simulink model "BlocoHidraulicoLAC_closeLoop"  (R2026a)
settings: Solver=ode15s  StopTime=5  FixedStep=0.001  MaxStep=1e-4
values from neighbouring files (symbols this model uses):
  Gamma = sys_d.B    [sintese_lqi_luenberger_lac.m]    (also in sintese_lqi_luenberger_lac_bateria_de_ensaio.m)
  K_i = -K_aug(3)    [sintese_lqi_luenberger_lac.m]    (also in sintese_lqi_luenberger_lac_bateria_de_ensaio.m)
  K_lqr = [K_pos, K_vel]    [sintese_lqi_luenberger_lac.m]    (also in sintese_lqi_luenberger_lac_bateria_de_ensaio.m)
  L_obs = place(Phi', Cx', polos_obs)'    [sintese_lqi_luenberger_lac.m]    (also in sintese_lqi_luenberger_lac_bateria_de_ensaio.m)
  Phi = sys_d.A    [sintese_lqi_luenberger_lac.m]    (also in sintese_lqi_luenberger_lac_bateria_de_ensaio.m)
undefined symbols (not defined in the file or in its folder): sigbuilder_block
(part 1 of 4)
settings Model: Creator=uidq5744  LastModifiedBy=uidq5744

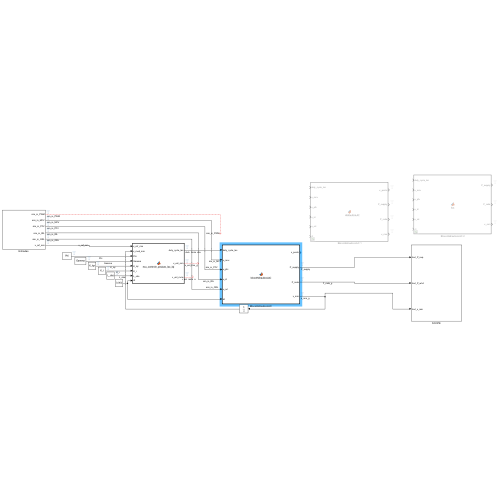
[thumbnail: Simulink's stored preview of the top-level diagram]
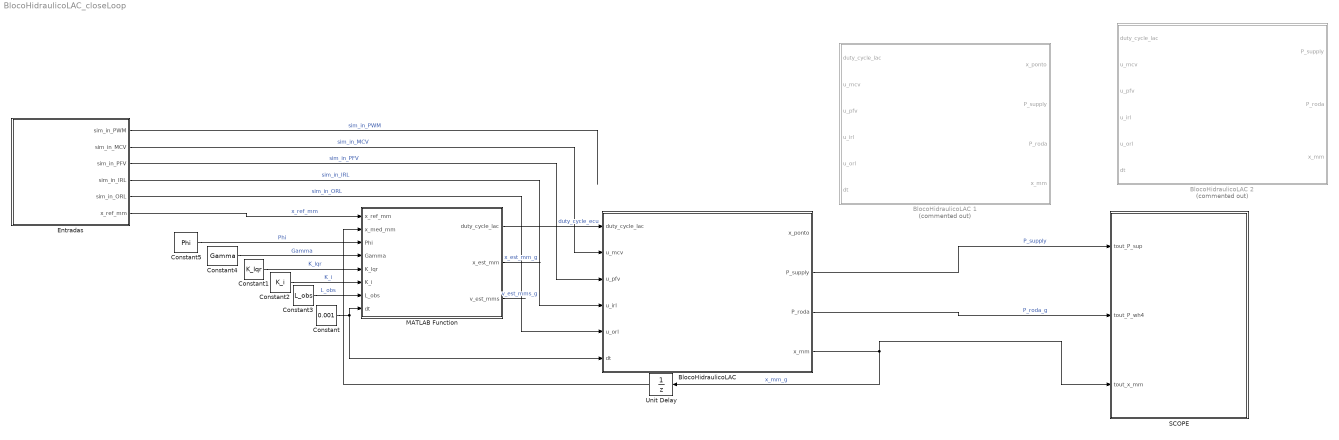
== system BlocoHidraulicoLAC_closeLoop ==
  " BlocoHidraulicoLAC " : MATLAB Function  TreatAsAtomicUnit=on
  " BlocoHidraulicoLAC 1" : MATLAB Function  Commented=on  TreatAsAtomicUnit=on
  " BlocoHidraulicoLAC 2" : MATLAB Function  Commented=on  TreatAsAtomicUnit=on
  Constant : Constant  Value=0.001
  Constant1 : Constant  Value=K_lqr
  Constant2 : Constant  Value=K_i
  Constant3 : Constant  Value=L_obs
  Constant4 : Constant  Value=Gamma
  Constant5 : Constant  Value=Phi
  "Entradas " : Subsystem
  MATLAB Function : MATLAB Function  TreatAsAtomicUnit=on
  SCOPE : Subsystem
  Unit Delay : UnitDelay  SampleTime=0.001
  wires:
  "Entradas "/4(sim_in_IRL) -> " BlocoHidraulicoLAC "/4(u_irl)  "sim_in_IRL"
  "Entradas "/5(sim_in_ORL) -> " BlocoHidraulicoLAC "/5(u_orl)  "sim_in_ORL"
  " BlocoHidraulicoLAC "/2(P_supply) -> SCOPE/1(tout_P_sup)  "P_supply"
  " BlocoHidraulicoLAC "/3(P_roda) -> SCOPE/2(tout_P_wh4)  "P_roda_g"
  Constant/1 -> MATLAB Function/8(dt), " BlocoHidraulicoLAC "/6(dt)
  " BlocoHidraulicoLAC "/4(x_mm) -> SCOPE/3(tout_x_mm), Unit Delay/1  "x_mm_g"
  "Entradas "/1(sim_in_PWM) -> ?  "sim_in_PWM"
  "Entradas "/2(sim_in_MCV) -> " BlocoHidraulicoLAC "/2(u_mcv)  "sim_in_MCV"
  "Entradas "/3(sim_in_PFV) -> " BlocoHidraulicoLAC "/3(u_pfv)  "sim_in_PFV"
  Unit Delay/1 -> MATLAB Function/2(x_med_mm)
  "Entradas "/6(x_ref_mm) -> MATLAB Function/1(x_ref_mm)  "x_ref_mm"
  Constant1/1 -> MATLAB Function/5(K_lqr)  "K_lqr"
  Constant2/1 -> MATLAB Function/6(K_i)  "K_i"
  Constant3/1 -> MATLAB Function/7(L_obs)  "L_obs"
  MATLAB Function/1(duty_cycle_lac) -> " BlocoHidraulicoLAC "/1(duty_cycle_lac)  "duty_cycle_ecu"
  Constant4/1 -> MATLAB Function/4(Gamma)  "Gamma"
  Constant5/1 -> MATLAB Function/3(Phi)  "Phi"
  MATLAB Function/2(x_est_mm) -> ?  "x_est_mm_g"
  MATLAB Function/3(v_est_mms) -> ?  "v_est_mms_g"

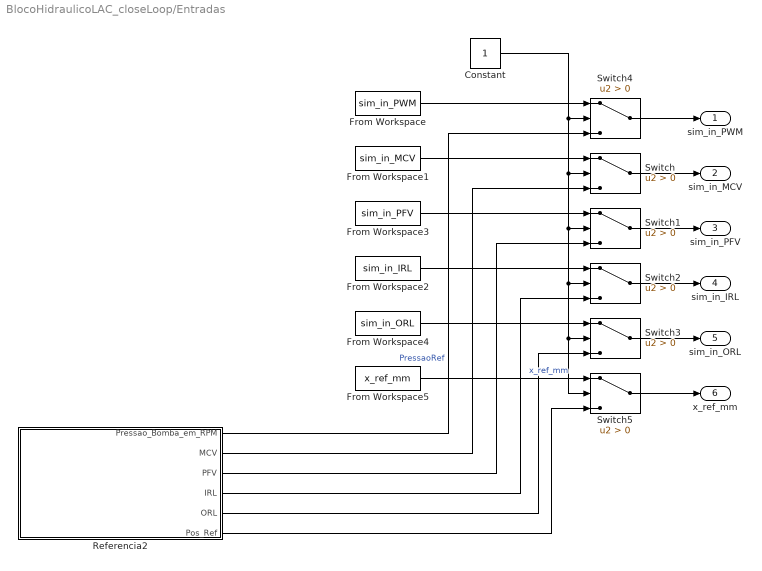
== system BlocoHidraulicoLAC_closeLoop/Entradas  ==
  Constant : Constant
  From Workspace : FromWorkspace  VariableName=sim_in_PWM
  From Workspace1 : FromWorkspace  VariableName=sim_in_MCV
  From Workspace2 : FromWorkspace  VariableName=sim_in_IRL
  From Workspace3 : FromWorkspace  VariableName=sim_in_PFV
  From Workspace4 : FromWorkspace  VariableName=sim_in_ORL
  From Workspace5 : FromWorkspace  VariableName=x_ref_mm
  Referencia2 : Subsystem  Tag=STV Subsys  LoadFcn=sigbuilder_block('load',[264 735 1440 846 ]);  StartFcn=sigbuilder_block('start');  StopFcn=sigbuilder_block('stop');  ClipboardFcn=sigbuilder_block('clipboard');  mask(Sigbuilder block){tuvar=[0:10]}
      mask help: Simulink:masks:SigbuilderBlock_MD
      mask init:
      | if ~strcmp(get_param(bdroot(gcbh),'SimulationStatus'),'stopped') tuvar = sigbuilder_block('maskInit'); end
      settings: CopyFcn=sigbuilder_block('copy');  DeleteFcn=sigbuilder_block('delete');  ModelCloseFcn=sigbuilder_block('modelClose');  PreSaveFcn=sigbuilder_block('preSave');  PauseFcn=sigbuilder_block('pause');  ContinueFcn=sigbuilder_block('continue');  NameChangeFcn=sigbuilder_block('namechange');  OpenFcn=sigbuilder_block('open',[323.25 1076.25 805.5 485.25 ]);  CloseFcn=sigbuilder_block('close');
      mask Display: plot(0, 0, 100, 100,[2, 2, 32, 32, 2], [68, 8, 8, 68, 68],[32, 2], [38, 38], [32, 19, 2],[53, 60, 44], [32, 17, 17, 2],[16, 16, 31, 31]);txt = getActiveGroup(gcbh);text(2, 100, txt,'verticalAlignment', 'top');
  Switch{,1..5} (6 alike) : Switch  Criteria=u2 > Threshold  SaturateOnIntegerOverflow=off  InputSameDT=off
  sim_in_PWM : Outport
  sim_in_MCV : Outport  Port=2
  sim_in_PFV : Outport  Port=3
  sim_in_IRL : Outport  Port=4
  sim_in_ORL : Outport  Port=5
  x_ref_mm : Outport  Port=6
  wires:
  Referencia2/1(Pressao_Bomba_em_RPM) -> Switch4/3  "PressaoRef"
  Referencia2/2(MCV) -> Switch/3
  Referencia2/4(IRL) -> Switch2/3
  Referencia2/3(PFV) -> Switch1/3
  Referencia2/5(ORL) -> Switch3/3
  Referencia2/6(Pos_Ref) -> Switch5/3
  From Workspace5/1 -> Switch5/1  "x_ref_mm"
  Switch3/1 -> sim_in_ORL/1
  Switch2/1 -> sim_in_IRL/1
  Switch1/1 -> sim_in_PFV/1
  Switch/1 -> sim_in_MCV/1
  Constant/1 -> Switch4/2, Switch/2, Switch1/2, Switch2/2, Switch3/2, Switch5/2
  From Workspace1/1 -> Switch/1
  From Workspace3/1 -> Switch1/1
  From Workspace2/1 -> Switch2/1
  From Workspace4/1 -> Switch3/1
  Switch4/1 -> sim_in_PWM/1
  From Workspace/1 -> Switch4/1
  Switch5/1 -> x_ref_mm/1

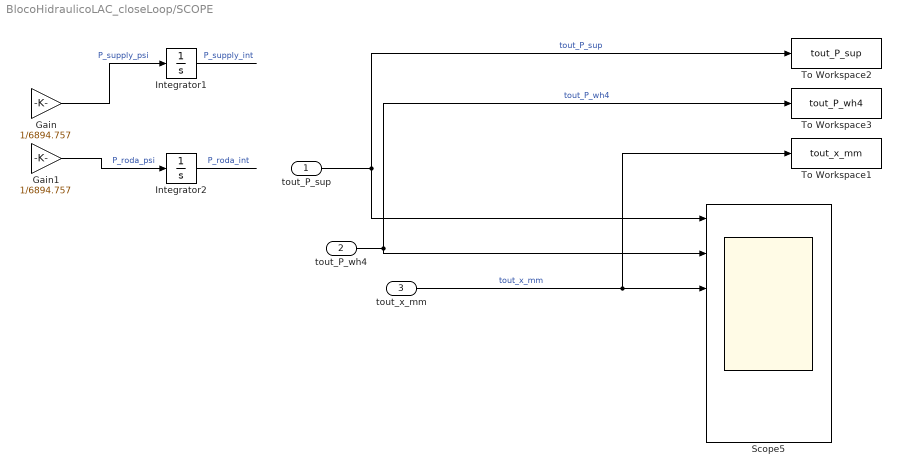
== system BlocoHidraulicoLAC_closeLoop/SCOPE ==
  tout_P_sup : Inport
  tout_P_wh4 : Inport  Port=2
  tout_x_mm : Inport  Port=3
  Gain : Gain  Gain=1/6894.757
  Gain1 : Gain  Gain=1/6894.757
  Integrator1 : Integrator
  Integrator2 : Integrator
  Scope5 : Scope  NumInputPorts=7
      settings: ActiveDisplayYMinimum=-5.7644121130531885E+294  ActiveDisplayYMaximum=5.18797090174787E+295  DataLoggingVariableName=ScopeData6
  To Workspace1 : ToWorkspace  VariableName=tout_x_mm  SaveFormat=Timeseries  SampleTime=-1
  To Workspace2 : ToWorkspace  VariableName=tout_P_sup  SaveFormat=Timeseries  SampleTime=-1
  To Workspace3 : ToWorkspace  VariableName=tout_P_wh4  SaveFormat=Timeseries  SampleTime=-1
  wires:
  tout_P_sup/1 -> Scope5/1, To Workspace2/1  "tout_P_sup"
  tout_P_wh4/1 -> Scope5/2, To Workspace3/1  "tout_P_wh4"
  tout_x_mm/1 -> To Workspace1/1, Scope5/3  "tout_x_mm"
  Gain1/1 -> Integrator2/1  "P_roda_psi"
  Gain/1 -> Integrator1/1  "P_supply_psi"
  Integrator2/1 -> ?  "P_roda_int"
  Integrator1/1 -> ?  "P_supply_int"

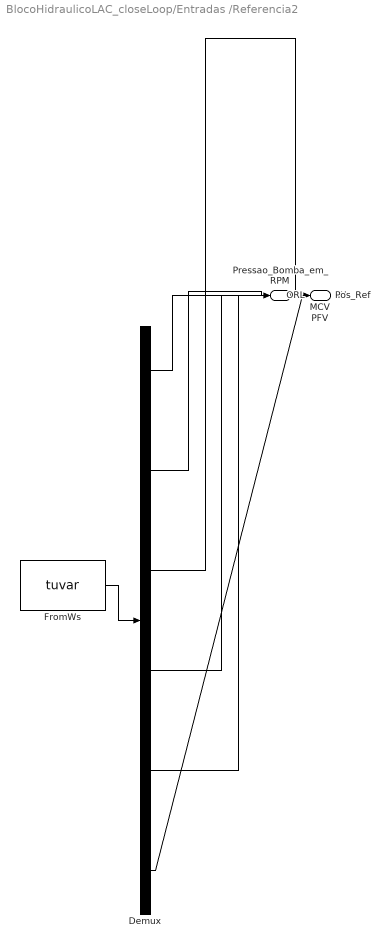
== system BlocoHidraulicoLAC_closeLoop/Entradas /Referencia2 ==
  Demux : Demux  Tag=STV Demux  Outputs=6
      settings: DisplayOption=none
  FromWs : FromWorkspace  Tag=STV FromWs  VariableName=tuvar
      SigBuilderData=|
      | common.afterFinalStr = 'Extrapolate'
      | common.sampleTime = 0
      | dataSet.timeRange = [0 50]
      | dataSet.name = 'Group 1'
      | sbobj.Groups.Name = 'Group 1'
      | sbobj.Groups.Signals(1).Name = 'Pressao_Bomba_em_RPM'
      | sbobj.Groups.Signals(1).XData = [0 1 1 1.995 2 3 3 4 4 48.3 48.3 50]
      | sbobj.Groups.Signals(1).YData = [0 0 100 100 200 200 50 50 0 0 30 85]
      | sbobj.Groups.Signals(2).Name = 'MCV'
      | sbobj.Groups.Signals(2).XData = [0 1 1 4 4 5.675 5.675 6.055 6.055 50]
      | sbobj.Groups.Signals(2).YData = [0 0 1 1 0 0 1 1 0 0]
      | sbobj.Groups.Signals(3).Name = 'PFV'
      | sbobj.Groups.Signals(3).XData = [0 1 1 4 4 5.635 5.635 6.575 6.575 50]
      | sbobj.Groups.Signals(3).YData = [0 0 1 1 0 0 1 1 0 0]
      | sbobj.Groups.Signals(4).Name = 'IRL'
      | sbobj.Groups.Signals(4).XData = [0 0.99 0.99 3.995 3.995 5.29 5.29 5.54 5.54 5.705 5.705 6.41 6.41 50]
      | sbobj.Groups.Signals(4).YData = [0 0 1 1 0 0 1 1 0 0 1 1 0 0]
      | sbobj.Groups.Signals(5).Name = 'ORL'
      | sbobj.Groups.Signals(5).XData = [0 4 4 4.5 4.5 15 20 50]
      | sbobj.Groups.Signals(5).YData = [0 0 1 1 0 0 0 0]
      | sbobj.Groups.Signals(6).Name = 'Pos_Ref'
      | sbobj.Groups.Signals(6).XData = [0 1 1 2 2 3 3 4 4 48.3 48.3 50]
      | sbobj.Groups.Signals(6).YData = [0 0 5 5 20 20 10 10 0 0 30 85]
      | sbobj.Groups.TimeRange = [0 50]
  Pressao_Bomba_em_RPM : Outport  Tag=STV Outport
  MCV : Outport  Tag=STV Outport  Port=2
  PFV : Outport  Tag=STV Outport  Port=3
  IRL : Outport  Tag=STV Outport  Port=4
  ORL : Outport  Tag=STV Outport  Port=5
  Pos_Ref : Outport  Tag=STV Outport  Port=6
  wires:
  Demux/1 -> Pressao_Bomba_em_RPM/1
  FromWs/1 -> Demux/1
  Demux/2 -> MCV/1
  Demux/3 -> PFV/1
  Demux/4 -> IRL/1
  Demux/5 -> ORL/1
  Demux/6 -> Pos_Ref/1

== matlab function BlocoHidraulicoLAC_closeLoop/ BlocoHidraulicoLAC  ==
  settings: updateMethod=DISCRETE
  data: x_ponto output; duty_cycle_lac input; u_mcv input; u_pfv input; u_irl input; u_orl input; P_supply output; P_roda output; dt input; x_mm output
function [x_ponto, P_supply, P_roda, x_mm] = blocoHidraulicoLAC(duty_cycle_lac, u_mcv, u_pfv, u_irl, u_orl, dt)
%#codegen
% =========================================================================
% BLOCO DE PLANTA FÍSICA HIDRO-MECÂNICA REVISADA (LAC + VÁLVULAS + CALIPER)
% =========================================================================
% Entradas:
%   duty_cycle_lac : Comando PWM de tensão/torque do motor [-100% a +100%]
%   u_mcv          : Sinal de acionamento da MCV (NA: 0 = Aberta, 1 = Fechada)
%   u_pfv          : Sinal de acionamento da PFV (NF: 0 = Fechada, 1 = Aberta)
%   u_irl          : Sinal de acionamento da IRL (NA: 0 = Aberta, 1 = Fechada)
%   u_orl          : Sinal de acionamento da ORL (NF: 0 = Fechada, 1 = Aberta)
%   dt             : Passo de amostragem numérico da simulação [s]
%
% Saídas:
%   x_ponto        : Velocidade linear instantânea do êmbolo [m/s]
%   P_supply       : Pressão de suprimento na câmara do LAC (Nó p1) [Pa]
%   P_roda         : Pressão na roda / caliper (Nó p3) [Pa]
%   x_mm           : Deslocamento linear do êmbolo do LAC [mm]
% =========================================================================

%% 1. PARÂMETROS FÍSICOS E GEOMÉTRICOS
rho       = 850.0;        % Densidade do fluido de freio [kg/m^3]
beta_eff  = 1.5e9;        % Bulk Modulus efetivo com microbolhas de ar [Pa]
A_lac     = 2.85e-4;      % Área da seção transversal do êmbolo [m^2]
V10       = 2.0e-5;       % Volume inicial da câmara de pressurização [m^3]
X_MAX     = 0.0537;       % Curso máximo de fim de curso [m] (53.7 mm)

% Mecânica do Motor DC, Fuso de Esferas e Carga Hidráulica
K_drv     = 0.085;        % Ganho de velocidade em vazio [m/s por unidade normalizada de duty]
tau_m     = 0.140;        % Constante de tempo eletromecânica do motor [s]
K_load    = 1.2e-5;       % Sensibilidade da velocidade contra a força de carga [m/(s*N)]

% Válvulas Solenoides e Orifícios
Cd        = 0.62;         % Coeficiente de descarga
A_max     = 3.5e-7;       % Área máxima de passagem dos orifícios [m^2]
tau_v     = 0.005;        % Constante de tempo eletrodinâmica do carretel [s]
pr        = 0.0;          % Pressão manométrica do reservatório [Pa]
dp_tol    = 2.0e3;        % Zona de regularização linear para fluxo de orifício [Pa]

% Compliance Hidráulica
C2        = 2.8e-12;      % Compliance da linha principal intermediária (Nó p2) [m^3/Pa]

%% 2. MEMÓRIA INTERNA DE ESTADOS (PERSISTENT)
persistent p1 p2 p3 x x_dot a_mcv a_pfv a_irl a_orl
if isempty(p1)
    p1    = 0.0;
    p2    = 0.0;
    p3    = 0.0;
    x     = 0.0;
    x_dot = 0.0;
    
    % Estados iniciais das aberturas das válvulas (0 a 1):
    a_mcv = 1.0; % MCV é Normalmente Aberta (NA)
    a_pfv = 0.0; % PFV é Normalmente Fechada (NF)
    a_irl = 1.0; % IRL é Normalmente Aberta (NA)
    a_orl = 0.0; % ORL é Normalmente Fechada (NF)
end

%% 3. DEFINIÇÃO DA SUB-INTEGRAÇÃO (PROTEÇÃO CONTRA RIGIDEZ NUMÉRICA)
dt_max_internal = 1.0e-5; % Passo interno máximo de 10 microssegundos
n_sub = ceil(dt / dt_max_internal);
if n_sub < 1
    n_sub = 1;
end
dt_sub = dt / double(n_sub);

%% 4. TARGETS DE ABERTURA DAS VÁLVULAS CONFORME TIPO FÍSICO
% MCV (NA): desenergizada (u=0) -> aberta (target=1); energizada (u=1) -> fecha (target=0)
target_mcv = 1.0 - double(u_mcv > 0.5);

% PFV (NF): desenergizada (u=0) -> fechada (target=0); energizada (u=1) -> abre (target=1)
target_pfv = double(u_pfv > 0.5);

% IRL (NA): desenergizada (u=0) -> aberta (target=1); energizada (u=1) -> fecha (target=0)
target_irl = 1.0 - double(u_irl > 0.5);

% ORL (NF): desenergizada (u=0) -> fechada (target=0); energizada (u=1) -> abre (target=1)
target_orl = double(u_orl > 0.5);

% Normalização e saturação do sinal de comando de PWM
u_norm = double(duty_cycle_lac) / 100.0;
u_norm = max(-1.0, min(1.0, u_norm));

%% 5. LOOP DE INTEGRAÇÃO TEMPORAL INTERNO
for k = 1:n_sub
    % 5.1 Dinâmica dos Carretéis das Válvulas (Filtro de 1ª ordem)
    a_mcv = a_mcv + (dt_sub / tau_v) * (-a_mcv + target_mcv);
    a_pfv = a_pfv + (dt_sub / tau_v) * (-a_pfv + target_pfv);
    a_irl = a_irl + (dt_sub / tau_v) * (-a_irl + target_irl);
    a_orl = a_orl + (dt_sub / tau_v) * (-a_orl + target_orl);

    % Saturação física das áreas (0 a 1)
    a_mcv = max(0.0, min(1.0, a_mcv));
    a_pfv = max(0.0, min(1.0, a_pfv));
    a_irl = max(0.0, min(1.0, a_irl));
    a_orl = max(0.0, min(1.0, a_orl));

    % Áreas efetivas instantâneas
    A_eff_mcv = a_mcv * A_max;
    A_eff_pfv = a_pfv * A_max;
    A_eff_irl = a_irl * A_max;
    A_eff_orl = a_orl * A_max;

    % 5.2 Diferenciais de Pressão
    dp_pfv = p1 - p2;
    dp_mcv = p2 - pr;
    dp_irl = p2 - p3;
    dp_orl = p3 - pr;

    % 5.3 Cálculo de Vazão dos Orifícios com Regularização Numérica Linear
    Q_pfv = fluxoOrificioRegularizado(Cd, A_eff_pfv, dp_pfv, rho, dp_tol);
    Q_mcv = fluxoOrificioRegularizado(Cd, A_eff_mcv, dp_mcv, rho, dp_tol);
    Q_irl = fluxoOrificioRegularizado(Cd, A_eff_irl, dp_irl, rho, dp_tol);
    Q_orl = fluxoOrificioRegularizado(Cd, A_eff_orl, dp_orl, rho, dp_tol);

    % 5.4 Modelo Eletromecânico Acoplado com Força Hidrostática Reversa
    F_hidro = p1 * A_lac; % Força axial contrária gerada pela pressão na câmara [N]
    
    % A velocidade-alvo do atuador decresce com a contra-pressão
    x_dot_alvo = (u_norm * K_drv) - (K_load * F_hidro);
    
    % Aceleração do conjunto fuso/motor
    x_ddot = (1.0 / tau_m) * (-x_dot + x_dot_alvo);

    % 5.5 Volume Residual da Câmara de Pressurização
    V1 = V10 - (A_lac * x);
    if V1 < 1.0e-7
        V1 = 1.0e-7; % Proteção contra volume nulo
    end

    % 5.6 Compliance Não Linear do Caliper C3(p3)
    % Em baixas pressões (folga de pastilha / air-gap), a compliance é alta.
    % % Acima de ~10 bar (1e6 Pa), o sistema atinge rigidez estrutural elevada.
    if p3 < 0.050 %1.0e6
        C3 = 2.5e-11; % Fase de pre-fill / absorção de curso
    else
        C3 = 8.267e-16; % Fase de deformação elástica do caliper
    end

    % % Limiar físico de encosto de pastilha: ~1.5 bar (1.5e5 Pa)
    % p_prefill = 1.5e5; 
    % if p3 < p_prefill
    %     C3 = 5.0e-12;       % Fase de absorção de folga
    % else
    %     C3 = 1.6e-12;       % Rigidez pós-encosto ajustada para o ensaio
    % end



    % 5.7 Derivadas de Pressão (Balanço de Massa Volumétrico)
    p1_dot = (beta_eff / V1) * (A_lac * x_dot - Q_pfv);
    p2_dot = (1.0 / C2)       * (Q_pfv - Q_mcv - Q_irl);
    p3_dot = (1.0 / C3)       * (Q_irl - Q_orl);

    % 5.8 Integração Temporal de Euler para os Estados
    x_dot = x_dot + x_ddot * dt_sub;
    x     = x     + x_dot  * dt_sub;

    % Batentes físicos do êmbolo mecânico
    if x >= X_MAX
        x = X_MAX;
        x_dot = min(0.0, x_dot);
    elseif x <= 0.0
        x = 0.0;
        x_dot = max(0.0, x_dot);
    end

    % Atualização das pressões com proteção contra cavitação manométrica
    p1 = max(0.0, p1 + p1_dot * dt_sub);
    p2 = max(0.0, p2 + p2_dot * dt_sub);
    p3 = max(0.0, p3 + p3_dot * dt_sub);
end

%% 6. ATRIBUIÇÃO DOS SINAIS DE SAÍDA DO BLOCO
x_ponto  = x_dot;
P_supply = p1/6894.757;
P_roda   = p3/6894.757;
x_mm     = x * 1000.0; % Conversão [m] -> [mm]

end

%% FUNÇÃO AUXILIAR LOCAL: VAZÃO EM ORIFÍCIO REGULARIZADA
function Q = fluxoOrificioRegularizado(Cd, A_eff, dp, rho, dp_tol)
%#codegen
abs_dp = abs(dp);
if abs_dp > dp_tol
    % Regime turbulento padrão de orifício
    Q = Cd * A_eff * sign(dp) * sqrt((2.0 / rho) * abs_dp);
else
    % Transição linear suave para eliminar derivada infinita em dp -> 0
    fator_linear = dp / dp_tol;
    Q = Cd * A_eff * fator_linear * sqrt((2.0 / rho) * dp_tol);
end
end
